simulink model "ThreephaseControl"  (R2024a)
settings: Solver=ode5  StartTime=0.0  StopTime=200  FixedStep=Ts  RelTol=1e-3  EnableMultiTasking=on
values from neighbouring files (symbols this model uses):
  Ts = 1e-4    (= 0.0001)    [params_tcst.m]
undefined symbols (not defined in the file or in its folder): Down, GPTRIP1SEL, GPTRIP2SEL, TZ1, TZ2, Up
libraries: c2802xlib x7, dspfdesign x1, spsPLL3phLib x1, mcbcontrolslib x1, eeTransforms x1, spsdq0toAlphaBetaZeroLib x1
settings Model: SimulationMode=external  ExtModeTrigDuration=8  Creator=omar_  LastModifiedBy=rodol
settings DataIOCC: LimitDataPoints=on  MaxDataPoints=1000000  SaveFormat=StructureWithTime  InspectSignalLogs=on
settings OptimizationCC: DefaultUnderspecifiedDataType=single  EnhancedBackFolding=on  PassReuseOutputArgsAs=Individual arguments  MaxStackSize=1024  OptimizeBlockOrder=speed  DifferentSizesBufferReuse=on  OptimizationCustomize=off  DenormalBehavior=FlushToZero  EfficientTunableParamExpr=on
settings DebuggingCC: ParameterTunabilityLossMsg=error  UnconnectedInputMsg=warning  UnconnectedOutputMsg=warning  UnconnectedLineMsg=warning
settings HardwareCC: ProdBitPerChar=16  ProdBitPerInt=16  ProdBitPerPointer=32  ProdBitPerSizeT=32  ProdBitPerPtrDiffT=32  ProdLargestAtomicInteger=Integer  ProdLargestAtomicFloat=None  ProdWordSize=16  ProdLongLongMode=on  ProdHWDeviceType=Texas Instruments->C2000
settings ModelReferenceCC: EnableRefExpFcnMdlSchedulingChecks=on
settings SFSimCC: MATLABDynamicMemAlloc=off
settings RTWCC: Description=Embedded Coder  SystemTargetFile=ert.tlc  HardwareBoard=TI Delfino F28379D LaunchPad  TemplateMakefile=ert_default_tmf  Toolchain=Texas Instruments Code Composer Studio (C2000)  CodeProfilingSaveOptions=MetricsOnly  GPUComputeCapability=3.5  DLArmComputeVersion=19.05
settings CodeAppCC: ForceParamTrailComments=on  IgnoreCustomStorageClasses=off  OperatorAnnotations=on  SimulinkDataObjDesc=on  SFDataObjDesc=on  InsertBlockDesc=on
settings ERTTargetCC: CodeReplacementLibrary=TI C28x  SupportContinuousTime=on  ExtMode=on  ExtModeTransport=4  ExtModeStaticAlloc=on  ExtModeAutomaticAllocSize=off  ExtModeStaticAllocSize=10000  ExtModeMexFile=ext_xcp  ExtModeMexArgs=1 6 5000000  ExtModeIntrfLevel=Level2 - Open

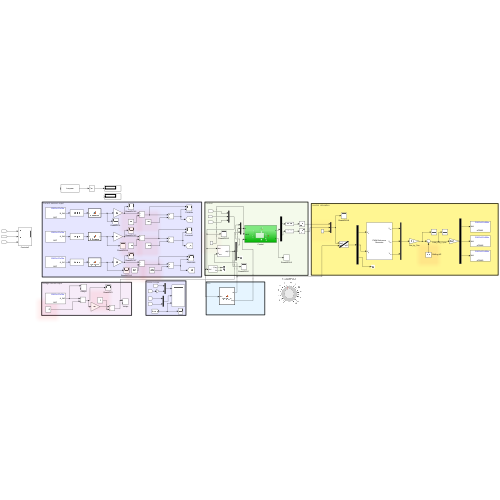
[thumbnail: Simulink's stored preview of the top-level diagram]
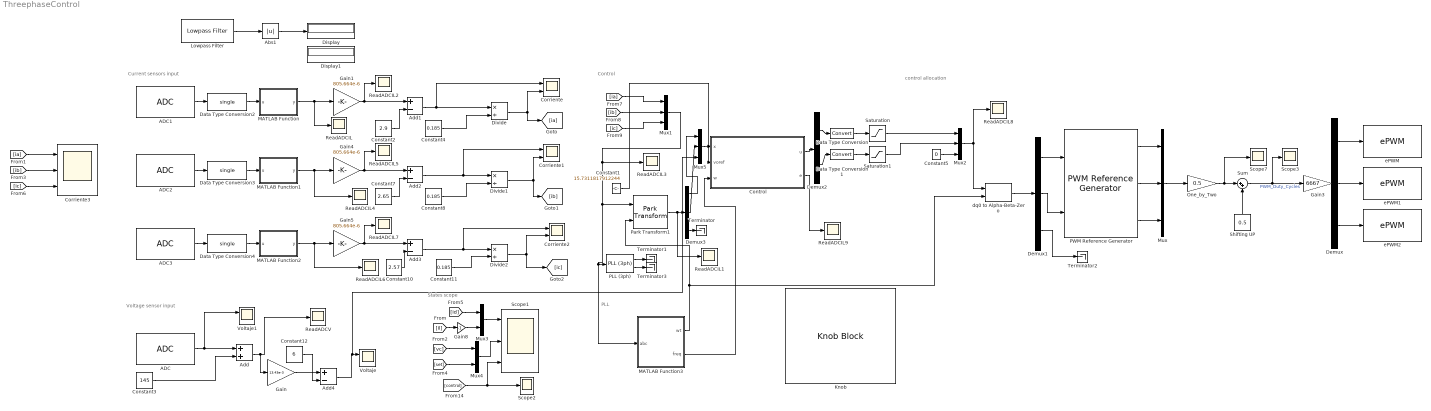
== system ThreephaseControl ==
  note: States scope
  note: Voltage sensor input
  note: Current sensors input
  note: control allocation
  note: Control
  note: PLL
  ADC : c2802xlib/ADC  blkParamProc=C2000_Type4  ADCModule=A  samplingMode=Single sample mode  ADCResolution=12-bit (Single-ended input)  useSOC1=SOC0  useSOC2=SOC0_SOC1  SOCAcquisitionWindow=15  SOCTriggerSource=Software  SOCInterruptTrigger=No ADCINT  Ts=Ts  dType=uint16  postInterrupt=off  interruptSel=ADCINT1  ADCINTContinuous=on  endma=off  chdma=1  conv1=ADCINA0  conv2=ADCINA0 and ADCINB0  conv1_Type4=ADCIN0  conv2_Type4=ADCIN0 and ADCIN1
  ADC1 : c2802xlib/ADC  blkParamProc=C2000_Type4  ADCModule=B  samplingMode=Single sample mode  ADCResolution=12-bit (Single-ended input)  useSOC1=SOC4  useSOC2=SOC0_SOC1  SOCAcquisitionWindow=15  SOCTriggerSource=Software  SOCInterruptTrigger=No ADCINT  Ts=Ts  dType=uint16  postInterrupt=off  interruptSel=ADCINT1  ADCINTContinuous=on  endma=off  chdma=1  conv1=ADCINA0  conv2=ADCINA0 and ADCINB0  conv1_Type4=ADCIN4  conv2_Type4=ADCIN0 and ADCIN1
  ADC2 : c2802xlib/ADC  blkParamProc=C2000_Type4  ADCModule=A  samplingMode=Single sample mode  ADCResolution=12-bit (Single-ended input)  useSOC1=SOC4  useSOC2=SOC0_SOC1  SOCAcquisitionWindow=15  SOCTriggerSource=Software  SOCInterruptTrigger=No ADCINT  Ts=Ts  dType=uint16  postInterrupt=off  interruptSel=ADCINT1  ADCINTContinuous=on  endma=off  chdma=1  conv1=ADCINA0  conv2=ADCINA0 and ADCINB0  conv1_Type4=ADCIN4  conv2_Type4=ADCIN0 and ADCIN1
  ADC3 : c2802xlib/ADC  blkParamProc=C2000_Type4  ADCModule=A  samplingMode=Single sample mode  ADCResolution=12-bit (Single-ended input)  useSOC1=SOC1  useSOC2=SOC0_SOC1  SOCAcquisitionWindow=15  SOCTriggerSource=Software  SOCInterruptTrigger=No ADCINT  Ts=Ts  dType=uint16  postInterrupt=off  interruptSel=ADCINT1  ADCINTContinuous=on  endma=off  chdma=1  conv1=ADCINA0  conv2=ADCINA0 and ADCINB0  conv1_Type4=ADCIN1  conv2_Type4=ADCIN0 and ADCIN1
  Abs1 : Abs  SaturateOnIntegerOverflow=off
  Add : Sum
  Add{1..4} (4 alike) : Sum  Inputs=+-
  Constant1 : Constant  Value=15.7311817912244  SampleTime=Ts
  Constant10 : Constant  Value=2.57  SampleTime=Ts
  Constant11 : Constant  Value=0.185  SampleTime=Ts
  Constant12 : Constant  Value=6  SampleTime=Ts
  Constant2 : Constant  Value=2.9  SampleTime=Ts
  Constant3 : Constant  Value=145  SampleTime=Ts
  Constant4 : Constant  Value=0.185  SampleTime=Ts
  Constant5 : Constant  Value=0  SampleTime=Ts
  Constant7 : Constant  Value=2.65  SampleTime=Ts
  Constant8 : Constant  Value=0.185  SampleTime=Ts
  Control : Subsystem
  Corriente : Scope  NumInputPorts=2
  Corriente1 : Scope  NumInputPorts=2
  Corriente2 : Scope  NumInputPorts=2
  Corriente3 : Scope  NumInputPorts=3
  Data Type Conversion : DataTypeConversion  SaturateOnIntegerOverflow=off  RndMeth=Floor
  Data Type Conversion1 : DataTypeConversion  SaturateOnIntegerOverflow=off  RndMeth=Floor
  Data Type Conversion2 : DataTypeConversion  OutDataTypeStr=single  SaturateOnIntegerOverflow=off  RndMeth=Floor
  Data Type Conversion3 : DataTypeConversion  OutDataTypeStr=single  SaturateOnIntegerOverflow=off  RndMeth=Floor
  Data Type Conversion4 : DataTypeConversion  OutDataTypeStr=single  SaturateOnIntegerOverflow=off  RndMeth=Floor
  Demux : Demux  Outputs=3
  Demux1 : Demux  Outputs=3
  Demux2 : Demux  Outputs=2
  Demux3 : Demux  Outputs=3
  Display : Display
  Display1 : Display
  Divide : Product  Inputs=*/
  Divide1 : Product  Inputs=*/
  Divide2 : Product  Inputs=*/
  Gain : Gain  Gain=13.43e-3  ParamDataTypeStr=double
  Gain1 : Gain  Gain=805.664e-6  ParamDataTypeStr=double
  Gain3 : Gain  Gain=6667
  Gain4 : Gain  Gain=805.664e-6  ParamDataTypeStr=double
  Gain5 : Gain  Gain=805.664e-6  ParamDataTypeStr=double
  Gain8 : Gain  Gain=-1
  Knob : KnobBlock  ScaleMax=35
  Lowpass Filter : dspfdesign/Lowpass Filter  FilterType=FIR  DesignForMinimumOrder=on  FilterOrder=8e3  PassbandFrequency=8e3  StopbandFrequency=12e3  PassbandRipple=0.1  StopbandAttenuation=80  SampleRateMode=Specify on dialog  SampleRate=44100  SimulateUsing=Interpreted execution  roundingMode=Floor  coeffsDataTypeStr=fixdt(1,16)
  MATLAB Function : MATLAB Function  TreatAsAtomicUnit=on
  MATLAB Function1 : MATLAB Function  TreatAsAtomicUnit=on
  MATLAB Function2 : MATLAB Function  TreatAsAtomicUnit=on
  MATLAB Function3 : MATLAB Function  TreatAsAtomicUnit=on
  Mux{,1..2,5} (4 alike) : Mux  Inputs=3
  Mux3 : Mux  Inputs=2
  Mux4 : Mux  Inputs=2
  One_by_Two : Gain  Gain=0.5  RndMeth=Simplest  OutDataTypeStr=Inherit: Same as input
  PLL (3ph) : spsPLL3phLib/PLL (3ph)  Fmin=45  Par_Init=[0, 60]  ParK=[180, 3200, 1]  TcD=1e-4  MaxRateChangeFreq=12  FilterCutOffFreq=25  Ts=0  AGC=on
  PWM Reference Generator : mcbcontrolslib/PWM Reference Generator  inSignal=Valphabeta  modType=SVM: space vector modulation
  Park Transform1 : eeTransforms/Park Transform  AxisAlignment=D-axis  PowerInvariant=off
  ReadADCIL{,1..9} (10 alike) : Scope
  ReadADCV : Scope
  Saturation : Saturate  UpperLimit=1  LowerLimit=-1
  Saturation1 : Saturate  UpperLimit=5  LowerLimit=-5
  Scope1 : Scope  NumInputPorts=3
  Scope2 : Scope
  Scope3 : Scope
  Scope7 : Scope
  Shifting UP : Constant  Value=0.5  SampleTime=Ts
  Sum : Sum  Inputs=|++
  Terminator{,1..3} (4 alike) : Terminator
  Voltaje : Scope  NumInputPorts=2
  Voltaje1 : Scope  NumInputPorts=2
  dq0 to Alpha-Beta-Zero : spsdq0toAlphaBetaZeroLib/dq0 to Alpha-Beta-Zero  Alignment=90 degrees behind phase A axis
  ePWM : c2802xlib/ePWM  PwmType=C2000_Type4  useModule=ePWM1  ePWMxLINKTBPRD=Not Linked  periodUnits=Clock cycles  timerSource=Specify via dialog  timerPeriod_clk=6667  timerPeriod_sec=0.0001  tbshadow=Counter equals to zero  countingMode=Up-Down  phaseActiveEnable=Set counter to phase value specified via dialog  phaseDirection=Count up after sync  phaseActive=0  synchronizationEnable=off  dcaevt1Sync=off  dcbevt1Sync=off  synchronizationOption=Counter equals to zero (CTR=Zero)  dcbevt1SyncOut=off  dcaevt1SyncOut=off  cmpdSyncOut=off  cmpcSyncOut=off  cmpbSyncOut=off  zeroSyncOut=off  swfSyncOut=off  perSynchronizationOption=Counter equals to period (CTR=PRD)  clockPrescale=1  HSclockPrescale=1  enswap=off  ePWMxAStatus=on  ePWMxAactionLogic1=Do nothing  ePWMxAactionLogic2=Do nothing  ePWMxAactionLogic3=Clear  ePWMxAactionLogic4=Set  ePWMxAactionLogic5=Do nothing  ePWMxAactionLogic6=Do nothing  ePWMxACSFenable=off  ePWMxACSFvalue=Forcing disable  ePWMxASFreload=Zero  ePWMxBStatus=on  ePWMxBactionLogic1=Do nothing  ePWMxBactionLogic2=Do nothing  ePWMxBactionLogic3=Do nothing  ePWMxBactionLogic4=Do nothing  ePWMxBactionLogic5=Do nothing  ePWMxBactionLogic6=Do nothing  ePWMxBCSFenable=off  ePWMxBCSFvalue=Forcing disable  ePWMxBSFreload=Zero  ePWNxBOutWay=on  ePWMxLINKCMPA=Not Linked  CMPAUnits=Clock cycles  CMPASource=Input port  CMPAValue_per=50  CMPAValue_clk=6667  enCMPAshadow=Counter equals to zero (CTR=Zero)  ePWMxLINKCMPB=Not Linked  CMPBUnits=Clock cycles  CMPBSource=Specify via dialog  CMPBValue_per=50  CMPBValue_clk=6667  enCMPBshadow=Counter equals to zero (CTR=Zero)  ePWMxLINKCMPC=Not Linked  CMPCUnits=Clock cycles  CMPCSource=Specify via dialog  CMPCValue_per=50  CMPCValue_clk=32000  enCMPCshadow=Counter equals to zero (CTR=Zero)  ePWMxLINKCMPD=Not Linked  CMPDUnits=Clock cycles  CMPDSource=Specify via dialog  CMPDValue_per=50  CMPDValue_clk=32000  enCMPDshadow=Counter equals to zero (CTR=Zero)  enableDBePWMxA=on  enableDBePWMxB=off  enhalfcycle=off  DBpolarity=Active high complementary (AHC)  DBedgeDelay=Positive  DBSource_ePWMxA=ePWMxA  DBSource_ePWMxB=ePWMxA  DBPeriodUnits=Seconds  DBperiodSource=Specify via dialog  REDperiod=0  FEDperiod=0  REDperiod_sec=0  FEDperiod_sec=10e-6  LoadModeDBRED=Immediate without using shadow  LoadModeDBFED=Immediate without using shadow  adcstartModuleA=on  adcrequestEventA=First event  adcstartEventA=Digital Compare Module A Event 1 start of conversion (DCAEVT1.soc)  adcstartEventA_type2=Counter equals to period (CTR=PRD)  adcstartModuleB=off  adcrequestEventB=First event  adcstartEventB=Counter equals to zero (CTR=Zero)  adcstartEventB_type2=Counter equals to zero (CTR=Zero)  intEn=off  intPrd=First event  intSel=Counter equals to zero (CTR=Zero)  intSel_type2=Counter equals to zero (CTR=Zero)  hrpe=off  enHRPWM=off  HRPWM_LoadMode=Counter equals to period (CTR=PRD)  HRPWM_CTLMode=Duty or Period control mode  HRPWM_EDGMode=Both edge  hrpeb=off  enHRPWMB=off  HRPWM_LoadModeB=Counter equals to zero (CTR=ZERO)  HRPWM_CTLModeB=Duty or Period control mode  HRPWM_EDGModeB=Both edge  enHRDBRED=off  enHRDBFED=off  enSFO=on  enautoconv=on  chopperEnable=off  chopperFrequency=1  chopperFirstwidth=1  chopperDuty=12.5%  tripZonesource=Specify via dialog  tzselOSHT1=off  tzselOSHT2=off  tzselOSHT3=off  tzselOSHT4=off  tzselOSHT5=off  tzselOSHT6=off  tzselOSHDCAEV1=off  tzselOSHDCBEV1=off  tzselCBC1=off  tzselCBC2=off  tzselCBC3=off  tzselCBC4=off  tzselCBC5=off  tzselCBC6=off  tzselCBCDCAEV2=off  tzselCBCDCBEV2=off  enTzOstIntr=off  enTzCbcIntr=off  enTzDCAEVT1Intr=off  enTzDCAEVT2Intr=off  enTzDCBEVT1Intr=off  enTzDCBEVT2Intr=off  tzclrCBCLatch=Counter equals to zero (CTR=Zero)  ePWMxAforced=No action  ePWMxBforced=No action  DCAEVT1forced=No action  DCBEVT1forced=No action  DCAEVT2forced=No action  DCBEVT2forced=No action  dcah=Trip Zone 1 input (TZ1)  dcal=Trip Zone 2 input (TZ2)  dcbh=Trip Zone 1 input (TZ1)  dcbl=Trip Zone 2 input (TZ2)  dcah_type2=GPTRIP1SEL/(TZ1)  dcal_type2=GPTRIP2SEL/(TZ2)  dcbh_type2=GPTRIP1SEL/(TZ1)  dcbl_type2=GPTRIP2SEL/(TZ2)  gendcaevt1=Event disabled  gendcaevt2=Event disabled  gendcbevt1=Event disabled  gendcbevt2=Event disabled  dcaevt1src=DCAEVT1 with sync  dcaevt2src=DCAEVT2 with sync  dcbevt1src=DCBEVT1 with sync  dcbevt2src=DCBEVT2 with sync  pulsesel=Counter equals to zero (CTR=Zero)  blankinv=off  blankoffset=0  blankwidth=0  evsrcsel=Filtered version of DCAEVT1 (DCAEVT1FILT)  encape=off
  ePWM1 : c2802xlib/ePWM  PwmType=C2000_Type4  useModule=ePWM2  ePWMxLINKTBPRD=Not Linked  periodUnits=Clock cycles  timerSource=Specify via dialog  timerPeriod_clk=6667  timerPeriod_sec=0.0001  tbshadow=Counter equals to zero  countingMode=Up-Down  phaseActiveEnable=Set counter to phase value specified via dialog  phaseDirection=Count up after sync  phaseActive=0  synchronizationEnable=off  dcaevt1Sync=off  dcbevt1Sync=off  synchronizationOption=Counter equals to zero (CTR=Zero)  dcbevt1SyncOut=off  dcaevt1SyncOut=off  cmpdSyncOut=off  cmpcSyncOut=off  cmpbSyncOut=off  zeroSyncOut=off  swfSyncOut=off  perSynchronizationOption=Counter equals to period (CTR=PRD)  clockPrescale=1  HSclockPrescale=1  enswap=off  ePWMxAStatus=on  ePWMxAactionLogic1=Do nothing  ePWMxAactionLogic2=Do nothing  ePWMxAactionLogic3=Clear  ePWMxAactionLogic4=Set  ePWMxAactionLogic5=Do nothing  ePWMxAactionLogic6=Do nothing  ePWMxACSFenable=off  ePWMxACSFvalue=Forcing disable  ePWMxASFreload=Zero  ePWMxBStatus=on  ePWMxBactionLogic1=Do nothing  ePWMxBactionLogic2=Do nothing  ePWMxBactionLogic3=Do nothing  ePWMxBactionLogic4=Do nothing  ePWMxBactionLogic5=Do nothing  ePWMxBactionLogic6=Do nothing  ePWMxBCSFenable=off  ePWMxBCSFvalue=Forcing disable  ePWMxBSFreload=Zero  ePWNxBOutWay=on  ePWMxLINKCMPA=Not Linked  CMPAUnits=Clock cycles  CMPASource=Input port  CMPAValue_per=50  CMPAValue_clk=6667  enCMPAshadow=Counter equals to zero (CTR=Zero)  ePWMxLINKCMPB=Not Linked  CMPBUnits=Clock cycles  CMPBSource=Specify via dialog  CMPBValue_per=50  CMPBValue_clk=6667  enCMPBshadow=Counter equals to zero (CTR=Zero)  ePWMxLINKCMPC=Not Linked  CMPCUnits=Clock cycles  CMPCSource=Specify via dialog  CMPCValue_per=50  CMPCValue_clk=32000  enCMPCshadow=Counter equals to zero (CTR=Zero)  ePWMxLINKCMPD=Not Linked  CMPDUnits=Clock cycles  CMPDSource=Specify via dialog  CMPDValue_per=50  CMPDValue_clk=32000  enCMPDshadow=Counter equals to zero (CTR=Zero)  enableDBePWMxA=on  enableDBePWMxB=off  enhalfcycle=off  DBpolarity=Active high complementary (AHC)  DBedgeDelay=Positive  DBSource_ePWMxA=ePWMxA  DBSource_ePWMxB=ePWMxA  DBPeriodUnits=Seconds  DBperiodSource=Specify via dialog  REDperiod=0  FEDperiod=0  REDperiod_sec=0  FEDperiod_sec=10e-6  LoadModeDBRED=Immediate without using shadow  LoadModeDBFED=Immediate without using shadow  adcstartModuleA=off  adcrequestEventA=First event  adcstartEventA=Digital Compare Module A Event 1 start of conversion (DCAEVT1.soc)  adcstartEventA_type2=Counter equals to period (CTR=PRD)  adcstartModuleB=off  adcrequestEventB=First event  adcstartEventB=Counter equals to zero (CTR=Zero)  adcstartEventB_type2=Counter equals to zero (CTR=Zero)  intEn=off  intPrd=First event  intSel=Counter equals to zero (CTR=Zero)  intSel_type2=Counter equals to zero (CTR=Zero)  hrpe=off  enHRPWM=off  HRPWM_LoadMode=Counter equals to period (CTR=PRD)  HRPWM_CTLMode=Duty or Period control mode  HRPWM_EDGMode=Both edge  hrpeb=off  enHRPWMB=off  HRPWM_LoadModeB=Counter equals to zero (CTR=ZERO)  HRPWM_CTLModeB=Duty or Period control mode  HRPWM_EDGModeB=Both edge  enHRDBRED=off  enHRDBFED=off  enSFO=on  enautoconv=on  chopperEnable=off  chopperFrequency=1  chopperFirstwidth=1  chopperDuty=12.5%  tripZonesource=Specify via dialog  tzselOSHT1=off  tzselOSHT2=off  tzselOSHT3=off  tzselOSHT4=off  tzselOSHT5=off  tzselOSHT6=off  tzselOSHDCAEV1=off  tzselOSHDCBEV1=off  tzselCBC1=off  tzselCBC2=off  tzselCBC3=off  tzselCBC4=off  tzselCBC5=off  tzselCBC6=off  tzselCBCDCAEV2=off  tzselCBCDCBEV2=off  enTzOstIntr=off  enTzCbcIntr=off  enTzDCAEVT1Intr=off  enTzDCAEVT2Intr=off  enTzDCBEVT1Intr=off  enTzDCBEVT2Intr=off  tzclrCBCLatch=Counter equals to zero (CTR=Zero)  ePWMxAforced=No action  ePWMxBforced=No action  DCAEVT1forced=No action  DCBEVT1forced=No action  DCAEVT2forced=No action  DCBEVT2forced=No action  dcah=Trip Zone 1 input (TZ1)  dcal=Trip Zone 2 input (TZ2)  dcbh=Trip Zone 1 input (TZ1)  dcbl=Trip Zone 2 input (TZ2)  dcah_type2=GPTRIP1SEL/(TZ1)  dcal_type2=GPTRIP2SEL/(TZ2)  dcbh_type2=GPTRIP1SEL/(TZ1)  dcbl_type2=GPTRIP2SEL/(TZ2)  gendcaevt1=Event disabled  gendcaevt2=Event disabled  gendcbevt1=Event disabled  gendcbevt2=Event disabled  dcaevt1src=DCAEVT1 with sync  dcaevt2src=DCAEVT2 with sync  dcbevt1src=DCBEVT1 with sync  dcbevt2src=DCBEVT2 with sync  pulsesel=Counter equals to zero (CTR=Zero)  blankinv=off  blankoffset=0  blankwidth=0  evsrcsel=Filtered version of DCAEVT1 (DCAEVT1FILT)  encape=off
  ePWM2 : c2802xlib/ePWM  PwmType=C2000_Type4  useModule=ePWM3  ePWMxLINKTBPRD=Not Linked  periodUnits=Clock cycles  timerSource=Specify via dialog  timerPeriod_clk=6667  timerPeriod_sec=0.0001  tbshadow=Counter equals to zero  countingMode=Up-Down  phaseActiveEnable=Set counter to phase value specified via dialog  phaseDirection=Count up after sync  phaseActive=0  synchronizationEnable=off  dcaevt1Sync=off  dcbevt1Sync=off  synchronizationOption=Counter equals to zero (CTR=Zero)  dcbevt1SyncOut=off  dcaevt1SyncOut=off  cmpdSyncOut=off  cmpcSyncOut=off  cmpbSyncOut=off  zeroSyncOut=off  swfSyncOut=off  perSynchronizationOption=Counter equals to period (CTR=PRD)  clockPrescale=1  HSclockPrescale=1  enswap=off  ePWMxAStatus=on  ePWMxAactionLogic1=Do nothing  ePWMxAactionLogic2=Do nothing  ePWMxAactionLogic3=Clear  ePWMxAactionLogic4=Set  ePWMxAactionLogic5=Do nothing  ePWMxAactionLogic6=Do nothing  ePWMxACSFenable=off  ePWMxACSFvalue=Forcing disable  ePWMxASFreload=Zero  ePWMxBStatus=on  ePWMxBactionLogic1=Do nothing  ePWMxBactionLogic2=Do nothing  ePWMxBactionLogic3=Do nothing  ePWMxBactionLogic4=Do nothing  ePWMxBactionLogic5=Do nothing  ePWMxBactionLogic6=Do nothing  ePWMxBCSFenable=off  ePWMxBCSFvalue=Forcing disable  ePWMxBSFreload=Zero  ePWNxBOutWay=on  ePWMxLINKCMPA=Not Linked  CMPAUnits=Clock cycles  CMPASource=Input port  CMPAValue_per=50  CMPAValue_clk=6667  enCMPAshadow=Counter equals to zero (CTR=Zero)  ePWMxLINKCMPB=Not Linked  CMPBUnits=Clock cycles  CMPBSource=Specify via dialog  CMPBValue_per=50  CMPBValue_clk=6667  enCMPBshadow=Counter equals to zero (CTR=Zero)  ePWMxLINKCMPC=Not Linked  CMPCUnits=Clock cycles  CMPCSource=Specify via dialog  CMPCValue_per=50  CMPCValue_clk=32000  enCMPCshadow=Counter equals to zero (CTR=Zero)  ePWMxLINKCMPD=Not Linked  CMPDUnits=Clock cycles  CMPDSource=Specify via dialog  CMPDValue_per=50  CMPDValue_clk=32000  enCMPDshadow=Counter equals to zero (CTR=Zero)  enableDBePWMxA=on  enableDBePWMxB=off  enhalfcycle=off  DBpolarity=Active high complementary (AHC)  DBedgeDelay=Positive  DBSource_ePWMxA=ePWMxA  DBSource_ePWMxB=ePWMxA  DBPeriodUnits=Seconds  DBperiodSource=Specify via dialog  REDperiod=0  FEDperiod=0  REDperiod_sec=0  FEDperiod_sec=10e-6  LoadModeDBRED=Immediate without using shadow  LoadModeDBFED=Immediate without using shadow  adcstartModuleA=off  adcrequestEventA=First event  adcstartEventA=Digital Compare Module A Event 1 start of conversion (DCAEVT1.soc)  adcstartEventA_type2=Counter equals to period (CTR=PRD)  adcstartModuleB=off  adcrequestEventB=First event  adcstartEventB=Counter equals to zero (CTR=Zero)  adcstartEventB_type2=Counter equals to zero (CTR=Zero)  intEn=off  intPrd=First event  intSel=Counter equals to zero (CTR=Zero)  intSel_type2=Counter equals to zero (CTR=Zero)  hrpe=off  enHRPWM=off  HRPWM_LoadMode=Counter equals to period (CTR=PRD)  HRPWM_CTLMode=Duty or Period control mode  HRPWM_EDGMode=Both edge  hrpeb=off  enHRPWMB=off  HRPWM_LoadModeB=Counter equals to zero (CTR=ZERO)  HRPWM_CTLModeB=Duty or Period control mode  HRPWM_EDGModeB=Both edge  enHRDBRED=off  enHRDBFED=off  enSFO=on  enautoconv=on  chopperEnable=off  chopperFrequency=1  chopperFirstwidth=1  chopperDuty=12.5%  tripZonesource=Specify via dialog  tzselOSHT1=off  tzselOSHT2=off  tzselOSHT3=off  tzselOSHT4=off  tzselOSHT5=off  tzselOSHT6=off  tzselOSHDCAEV1=off  tzselOSHDCBEV1=off  tzselCBC1=off  tzselCBC2=off  tzselCBC3=off  tzselCBC4=off  tzselCBC5=off  tzselCBC6=off  tzselCBCDCAEV2=off  tzselCBCDCBEV2=off  enTzOstIntr=off  enTzCbcIntr=off  enTzDCAEVT1Intr=off  enTzDCAEVT2Intr=off  enTzDCBEVT1Intr=off  enTzDCBEVT2Intr=off  tzclrCBCLatch=Counter equals to zero (CTR=Zero)  ePWMxAforced=No action  ePWMxBforced=No action  DCAEVT1forced=No action  DCBEVT1forced=No action  DCAEVT2forced=No action  DCBEVT2forced=No action  dcah=Trip Zone 1 input (TZ1)  dcal=Trip Zone 2 input (TZ2)  dcbh=Trip Zone 1 input (TZ1)  dcbl=Trip Zone 2 input (TZ2)  dcah_type2=GPTRIP1SEL/(TZ1)  dcal_type2=GPTRIP2SEL/(TZ2)  dcbh_type2=GPTRIP1SEL/(TZ1)  dcbl_type2=GPTRIP2SEL/(TZ2)  gendcaevt1=Event disabled  gendcaevt2=Event disabled  gendcbevt1=Event disabled  gendcbevt2=Event disabled  dcaevt1src=DCAEVT1 with sync  dcaevt2src=DCAEVT2 with sync  dcbevt1src=DCBEVT1 with sync  dcbevt2src=DCBEVT2 with sync  pulsesel=Counter equals to zero (CTR=Zero)  blankinv=off  blankoffset=0  blankwidth=0  evsrcsel=Filtered version of DCAEVT1 (DCAEVT1FILT)  encape=off
  wires:
  Demux3/3 -> Terminator/1
  [control] -> Scope2/1, Scope1/3
  [il] -> Gain8/1
  [set] -> Mux4/2
  Gain8/1 -> Mux3/2
  [vc] -> Mux4/1
  Mux3/1 -> Scope1/1
  [id] -> Mux3/1
  Mux4/1 -> Scope1/2
  Data Type Conversion/1 -> Saturation/1
  Data Type Conversion1/1 -> Saturation1/1
  Saturation/1 -> Mux2/1
  Saturation1/1 -> Mux2/2
  Constant5/1 -> Mux2/3
  Gain3/1 -> Demux/1
  Demux/2 -> ePWM1/1
  Demux/1 -> ePWM/1
  Sum/1 -> Gain3/1, Scope3/1  "PWM_Duty_Cycles"
  Shifting UP/1 -> Sum/2
  One_by_Two/1 -> Sum/1, Scope7/1
  Demux/3 -> ePWM2/1
  Demux1/1 -> PWM Reference Generator/1
  Demux1/2 -> PWM Reference Generator/2
  PWM Reference Generator/1 -> Mux/1
  PWM Reference Generator/2 -> Mux/2
  PWM Reference Generator/3 -> Mux/3
  Mux/1 -> One_by_Two/1
  dq0 to Alpha-Beta-Zero/1 -> Demux1/1
  Constant2/1 -> Add1/2
  Add1/1 -> Divide/1, Corriente/1
  Add/1 -> ReadADCV/1, Gain/1
  ADC/1 -> Add/1, Voltaje1/1
  Constant3/1 -> Add/2
  Gain/1 -> Add4/1
  Add4/1 -> Mux5/3, Voltaje/1
  Gain1/1 -> Add1/1, ReadADCIL2/1
  Abs1/1 -> Display/1
  Constant4/1 -> Divide/2
  Divide/1 -> [ia], Corriente/2
  MATLAB Function/1(y) -> ReadADCIL/1, Gain1/1
  Mux1/1 -> MATLAB Function3/1(abc), PLL (3ph)/1, Park Transform1/1, ReadADCIL3/1
  ADC1/1 -> Data Type Conversion2/1
  Data Type Conversion2/1 -> MATLAB Function/1(u)
  Lowpass Filter/1 -> Abs1/1
  Park Transform1/1 -> ReadADCIL1/1, Demux3/1
  ADC2/1 -> Data Type Conversion3/1
  MATLAB Function1/1(y) -> ReadADCIL4/1, Gain4/1
  Gain4/1 -> Add2/1, ReadADCIL5/1
  Data Type Conversion3/1 -> MATLAB Function1/1(u)
  Constant7/1 -> Add2/2
  Add2/1 -> Divide1/1, Corriente1/1
  Constant8/1 -> Divide1/2
  Divide1/1 -> Corriente1/2, [ib]
  ADC3/1 -> Data Type Conversion4/1
  MATLAB Function2/1(y) -> ReadADCIL6/1, Gain5/1
  Gain5/1 -> Add3/1, ReadADCIL7/1
  Data Type Conversion4/1 -> MATLAB Function2/1(u)
  Constant10/1 -> Add3/2
  Add3/1 -> Divide2/1, Corriente2/1
  Constant11/1 -> Divide2/2
  Divide2/1 -> Corriente2/2, [ic]
  [ib] -> Corriente3/2
  [ia] -> Corriente3/1
  [ic] -> Corriente3/3
  Constant12/1 -> Add4/2
  Demux2/1 -> Data Type Conversion/1
  Demux2/2 -> Data Type Conversion1/1
  Control/1(u) -> Demux2/1
  Mux5/1 -> Control/1(x)
  Demux3/1 -> Mux5/1
  Demux3/2 -> Mux5/2
  Constant1/1 -> Control/2(voref)
  [ia] -> Mux1/1
  [ib] -> Mux1/2
  [ic] -> Mux1/3
  Mux2/1 -> dq0 to Alpha-Beta-Zero/1, ReadADCIL8/1
  Control/2(e) -> ReadADCIL9/1
  PLL (3ph)/1 -> Terminator1/1
  Demux1/3 -> Terminator2/1
  MATLAB Function3/2(freq) -> Control/3(w)
  PLL (3ph)/2 -> Terminator3/1
  MATLAB Function3/1(wt) -> dq0 to Alpha-Beta-Zero/2, Park Transform1/2

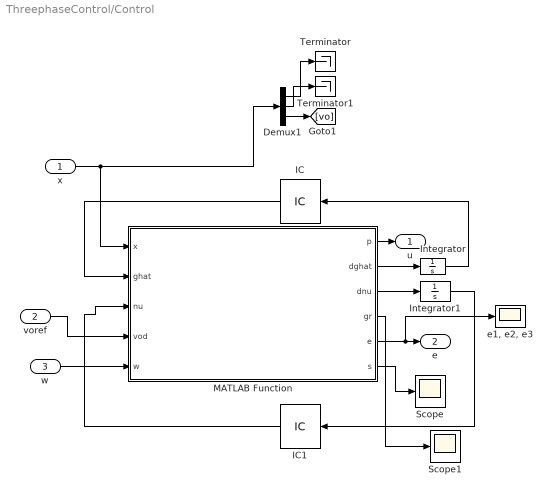
== system ThreephaseControl/Control ==
  x : Inport
  voref : Inport  Port=2
  w : Inport  Port=3
  Demux1 : Demux  Outputs=3
  IC : InitialCondition
  IC1 : InitialCondition
  Integrator : Integrator
  Integrator1 : Integrator
  MATLAB Function : MATLAB Function  TreatAsAtomicUnit=on
  Scope : Scope
  Scope1 : Scope
  Terminator : Terminator
  Terminator1 : Terminator
  "e1, e2, e3" : Scope
  u : Outport
  e : Outport  Port=2
  wires:
  x/1 -> MATLAB Function/1(x), Demux1/1
  Demux1/3 -> [vo]
  Demux1/1 -> Terminator/1
  Demux1/2 -> Terminator1/1
  MATLAB Function/1(p) -> u/1
  MATLAB Function/2(dghat) -> Integrator/1
  Integrator/1 -> IC/1
  MATLAB Function/3(dnu) -> Integrator1/1
  IC/1 -> MATLAB Function/2(ghat)
  Integrator1/1 -> IC1/1
  IC1/1 -> MATLAB Function/3(nu)
  MATLAB Function/5(e) -> "e1, e2, e3"/1, e/1
  voref/1 -> MATLAB Function/4(vod)
  MATLAB Function/6(s) -> Scope/1
  MATLAB Function/4(gr) -> Scope1/1
  w/1 -> MATLAB Function/5(w)

== matlab function ThreephaseControl/MATLAB Function3 ==
  data: abc input; wt output; freq output; PL parameter
function [wt, freq] = spll3ph_srf(abc, PL)
%SPLL3PH_SRF  Three-phase synchronous-reference-frame PLL, discrete.
%   Same structure as TI C2000Ware SPLL_3PH_SRF (spll_3ph_srf.h):
%     v_q -> PI loop filter (Tustin, coefficients b0, b1) -> fo = fn + ylf [Hz]
%     -> theta(k) = theta(k-1) + 2*pi*fo*Ts, wrapped to [0, 2*pi).
%   The input vector is normalized, so the loop gain does not depend on its
%   amplitude (TI expects per-unit voltages).
%
%   Inputs
%     abc = [a; b; c]  synchronizing three-phase signal (voltages or currents)
%     PL  = parameter struct (MATLAB Function "Parameter", non-tunable):
%           PL.fn      nominal frequency [Hz]          (e.g. 446)
%           PL.Ts      sample time [s]                 (1e-4)
%           PL.Kp, PL.Ki  PI gains, output in Hz       (see spll_gains below)
%           PL.ylfmax  max frequency deviation [Hz]    (TI uses 200)
%           PL.minmag  min |x_alphabeta| to update     (e.g. 0.05)
%
%   Outputs
%     wt   = estimated angle theta in [0, 2*pi) [rad], d axis aligned with abc
%     freq = estimated frequency fo [Hz]  (w = 2*pi*freq for ctrl16)
%
%   Block settings: discrete, Sample time = PL.Ts.

persistent theta ylf vq1
if isempty(theta)
    theta = 0;  ylf = 0;  vq1 = 0;
end

% Clarke, amplitude invariant (three-wire)
xa = abc(1);
xb = (abc(1) + 2*abc(2))/sqrt(3);

% Park with the current angle; q component of the normalized vector
mag = sqrt(xa^2 + xb^2);
if mag > PL.minmag
    vq = (-xa*sin(theta) + xb*cos(theta))/mag;     % = sin(theta_x - theta)
else
    vq = 0;                                       % free-running at fn
end

% Loop filter (TI form): ylf(k) = ylf(k-1) + b0*vq(k) + b1*vq(k-1)
b0 =  PL.Kp + PL.Ki*PL.Ts/2;
b1 = -PL.Kp + PL.Ki*PL.Ts/2;
ylf = ylf + b0*vq + b1*vq1;
ylf = min(max(ylf, -PL.ylfmax), PL.ylfmax);
vq1 = vq;

% VCO
freq  = PL.fn + ylf;
theta = theta + 2*pi*freq*PL.Ts;
if theta >= 2*pi, theta = theta - 2*pi; end
if theta < 0,     theta = theta + 2*pi; end

wt = theta;
end

== matlab function ThreephaseControl/MATLAB Function ==
  data: u input; y output
function y = iir_lowpass(u)
    % Parámetros del filtro
    persistent x z a b;
    Fs = 10000; % Frecuencia de muestreo
    Fc = 700;  % Frecuencia de corte
    if isempty(x)
        % Coeficientes del filtro Butterworth orden 2
        [b, a] = butter(2, Fc / (Fs / 2)); 
        x = zeros(2, 1); % Estados de entrada anteriores
        z = zeros(2, 1); % Estados de salida anteriores
    end

    % Aplicar el filtro (forma directa II transpuesta)
    y = b(1)*u + x(1);
    x(1) = b(2)*u - a(2)*y + x(2);
    x(2) = b(3)*u - a(3)*y;

end

== matlab function ThreephaseControl/MATLAB Function1 ==
  data: u input; y output
function y = iir_lowpass(u)
    % Parámetros del filtro
    persistent x z a b;
    Fs = 10000; % Frecuencia de muestreo
    Fc = 1800;  % Frecuencia de corte
    if isempty(x)
        % Coeficientes del filtro Butterworth orden 2
        [b, a] = butter(2, Fc / (Fs / 2)); 
        x = zeros(2, 1); % Estados de entrada anteriores
        z = zeros(2, 1); % Estados de salida anteriores
    end

    % Aplicar el filtro (forma directa II transpuesta)
    y = b(1)*u + x(1);
    x(1) = b(2)*u - a(2)*y + x(2);
    x(2) = b(3)*u - a(3)*y;

end

== matlab function ThreephaseControl/MATLAB Function2 ==
  data: u input; y output
function y = iir_lowpass(u)
    % Parámetros del filtro
    persistent x z a b;
    Fs = 10000; % Frecuencia de muestreo
    Fc = 1000;  % Frecuencia de corte
    if isempty(x)
        % Coeficientes del filtro Butterworth orden 2
        [b, a] = butter(2, Fc / (Fs / 2)); 
        x = zeros(2, 1); % Estados de entrada anteriores
        z = zeros(2, 1); % Estados de salida anteriores
    end

    % Aplicar el filtro (forma directa II transpuesta)
    y = b(1)*u + x(1);
    x(1) = b(2)*u - a(2)*y + x(2);
    x(2) = b(3)*u - a(3)*y;

end

== matlab function ThreephaseControl/Control/MATLAB Function ==
  data: x input; p output; ghat input; nu input; vod input; w input; dghat output; dnu output; gr output; e output; s output; P parameter
function [p, dghat, dnu, gr, e, s] = ctrl16(x, ghat, nu, vod, w, P)
%CTRL16  Adaptive passivity-based controller, law (16) of TCST 26-1303.
%
%   Inputs
%     x     = [id; iq; vo]  measured dq currents [A] and dc-link voltage [V]
%     ghat  = conductance estimate [S]      (state, integrate dghat outside)
%     nu    = filtered voltage error [V]    (state, integrate dnu outside)
%     vod   = dc-link voltage reference [V]
%     w     = source angular frequency [rad/s] (= 2*pi*Freq from the PLL)
%     P     = parameter struct (see params_tcst.m), MATLAB Function
%             "Parameter" data, non-tunable
%
%   Outputs
%     p     = [pd; pq]  saturated modulation indices, p in S = [-ad,ad]x[-aq,aq]
%     dghat = time derivative of ghat, projected update (16d)
%     dnu   = time derivative of nu, first-order filter (16c)
%     gr    = reference conductance (16c) [S]
%     e     = [e1; e2; e3] errors (6)
%     s     = passive-output component s = I(gr) e3 - vod e1, see (9)
%
%   Notation and equation numbers follow the revised manuscript.

id = x(1);  iq = x(2);  vo = x(3);

% ---- Reference conductance (16c) ---------------------------------------
gr = ghat - P.kappa*P.nubar*tanh(nu/P.nubar);

% ---- Equilibrium current and feedforward, Eqs. (2) and (4) -------------
Ir   = eqCurrent(gr, vod, P);
pdeq =  2*(P.Em - P.R*Ir)/vod;
pqeq = -2*P.L*w*Ir/vod;

% ---- Errors (6) and passive output (9) ---------------------------------
e1 = id - Ir;
e2 = iq;
e3 = vo - vod;
s  = Ir*e3 - vod*e1;

% ---- Channel-wise saturated port law (16a)-(16b) -----------------------
pd = sat(pdeq - (2*P.ks/3)*s,        P.ad);
pq = sat(pqeq + (2*P.kq/(3*vod))*iq, P.aq);
p  = [pd; pq];

% ---- Filter (16c) and projected estimator (16d) ------------------------
dnu   = P.lambdaf*(e3 - nu);
y     = -2*P.gamma*vod*e3 - P.gamma*P.sigma*(ghat - P.gc);
dghat = proj(ghat, y, P.glow, P.gup, P.epsp);

e = [e1; e2; e3];
end

% =========================================================================
function I = eqCurrent(g, vod, P)
% Smaller root of the power balance (3), Eq. (4). The argument of sqrt is
% positive whenever g < gmax, which (17) guarantees on Gr; it is clipped
% only to protect the simulation if (17) is violated.
arg = P.Em^2 - (8/3)*P.R*vod^2*g;
I   = (P.Em - sqrt(max(arg, 0)))/(2*P.R);
end

function v = sat(u, a)
% Saturation onto [-a, a].
v = min(max(u, -a), a);
end

function py = proj(g, y, glow, gup, ep)
% Smooth projection (14): keeps g in [glow-ep, gup+ep].
cp = min(1, max(0, (g - gup)/ep));
cm = min(1, max(0, (glow - g)/ep));
py = y - cp*max(y, 0) - cm*min(y, 0);
end
